simulink model "vdynblksskidpad_final"  (R2026b)
settings: Solver=ode23t  StopTime=inf  RelTol=5e-3
model workspace (MAT data in the model file):
  Eng.Tbts = [18.9199441202 18.9199441202 24.2934146345 29.2101064979 38.0525747067 43.75 43.7497238015 43.7499913003 43.75 43.75 43.75 43.75 43.75 39.375 35 30.625]
  Eng.Nbts = [0 1500 2107.14285714 2714.28571429 3321.42857143 3928.57142857 4535.71428571 5142.85714286 5750 6357.14285714 6964.28571429 7571.42857143 8178.57142857 8785.71428571 9392.85714286 10000]
  Nmtr = 11.5
  StartupTrim.BodyZ = -0.297506277079
  StartupTrim.Pitch = 0.00303068622905
  StartupTrim.TireCompression = 0.010016854716
  StartupTrim.WheelRadius = [0.290736809479 0.290736800352 0.290650131428 0.290650124633]
  SteerLim = 60
  TrackPoints = [-15 -12 -9 -6 -3 5.58745102111e-16 2.81978007367 5.36354042717 7.38228007367 8.67839071119 9.125 8.67839071119 ... (270 elements, 90x3)]
  Trans.InputShaftInertia = 0.01
  Trans.InputShaftDamping = 0.001
  Trans.FinalDrive = 3.25
  Trans.GearRatios = [-3.82 4.56 4.56 3.385 2.857 2.444 2 1]
  Trans.GearNums = [-1 0 1 2 3 4 5 6]
  Trans.Inertias = [0.032 0.007 0.032 0.025 0.0155 0.007 0.0025 0.0025]
  Trans.DampingCoeffs = [0.003 0.001 0.003 0.0025 0.002 0.001 0.001 0.001]
  Trans.Efficiencies = [0.9 0.9 0.9 0.9 0.9 0.95 0.95 0.95]
  Trans.ShiftTau = 0.02
  Ts = 0.02
  VEH.Mass = 230
  VEH.StaticNormalFrontLoad.FR = 575
  VEH.StaticNormalFrontLoad.FL = 575
  VEH.StaticNormalRearLoad.RR = 575
  VEH.StaticNormalRearLoad.RL = 322
  VEH.WheelBase = 1.7
  VEH.FrontAxlePositionfromCG = 0.75
  VEH.RearAxlePositionfromCG = 0.75
  VEH.HeightCG = 0.25
  VEH.FrontalArea = 2.11
  VEH.DragCoefficient = 0.33
  VEH.NumberOfWheelsPerAxle = 2
  VEH.PitchMomentInertia = 384.533333333
  VEH.RollMomentInertia = 86.4666666667
  VEH.YawMomentInertia = 413.2
  VEH.SteeringRatio = 18
  VEH.TrackWidth = 1.2
  VEH.SprungMass = 210
  VEH.InitialLongPosition = -15
  VEH.InitialLatPosition = 0
  VEH.InitialVertPosition = -0.2
  VEH.InitialRollAngle = 0
  VEH.InitialPitchAngle = 0
  VEH.InitialYawAngle = 0
  VEH.InitialLongVel = 0
  VEH.InitialLatVel = 0
  VEH.InitialVertVel = 0
  VEH.InitialRollRate = 0
  VEH.InitialPitchRate = 0
  VEH.InitialYawRate = 0
values from neighbouring files (symbols this model uses):
  n = size(e.Data,2)    [plot_skidpad_signals.m]
  z = tsMatrix(out.diagWheel.z)    [skidpad_settle_start.m]
undefined symbols (not defined in the file or in its folder): BdyFrm, InertFrm, magnitude
libraries: autolibsharedcoupling x11, simulink x8, sim3dlib x7, autolibshareddiff x5, autolibutils x4, sim3dautolib x3, vehdynlibtirecommon x3, sharedtransform x3, vehdynlibdriver x2, vehdynlibsteering x2, vehdynlibeom x2, vehdynlibviscommon x2
(part 1 of 5)
settings Model: Creator=The MathWorks, Inc.  LastModifiedBy=aaditya
settings SolverCC: ZeroCrossAlgorithm=Adaptive
settings OptimizationCC: ReuseModelBlockBuffer=off
settings DebuggingCC: IgnoredZcDiagnostic=none  SubsystemReferenceDiagnosticForUnitTest=warning

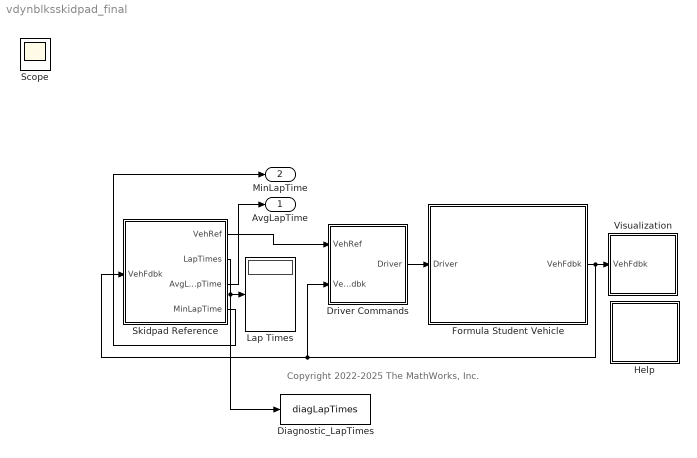
== system vdynblksskidpad_final ==
  note: Copyright 2022-2025 The MathWorks, Inc.
  Diagnostic_LapTimes : ToWorkspace  VariableName=diagLapTimes  SaveFormat=Timeseries  SampleTime=0.01
  Driver Commands : Subsystem  VariantControl=0
      mask Display: image('driverlatlongshift.png');
  Formula Student Vehicle : Subsystem  Variant=on  VariantControl=Choice  mask(Vehicle Setup){vehType=Simulink Physics}
      mask prompts: vehType "Vehicle Type:"
      mask help:
      | Choose a vehicle with powertrain and vehicle physics from Simulink blocks or one that uses a game engine physics.
      | The model will automatically configure the subsystems and settings to accomodate your choice.
      mask Help: eval('vdynblkshelp(''vdynblksformula'')');
      mask TypeOptions vehType: Game Engine Physics | Simulink Physics
      mask Callback vehType:
      | if strcmp(get_param(gcb,"vehType"),"Game Engine Physics")
      |     set_param([bdroot(gcs) '/Visualization/3D Visualization'],'engine3D','Enabled - Game Physics Vehicle')
      | else
      |     if strcmp(get_param([bdroot(gcs) '/Visualization/3D Visualization'],'engine3D'),'Enabled - Game Physics Vehicle')
      |         set_param([bdroot(gcs) '/Visualization/3D Visualization'],'engine3D','Enabled - Simulink 3D Vehicle')
      |     end
      | end
      mask Display: image('$imagefile'); % Use "Edit Image" on toolstrip to change.
  Help : Subsystem
      settings: OpenFcn=eval('vdynblkshelp(''vdynblksformula'')');
      mask Display: disp('Help')
  Lap Times : Display
  Skidpad Reference : Subsystem
      mask Display:
      | entryWidth = 3.453;
      | hOffset = 40;
      | vOffset = 15;
      | offset = [40,15];
      | entryConesLocR = [entryWidth/2 -12; entryWidth/2 -7.939];
      | entryConesLocL = [-entryWidth/2 -12;-entryWidth/2 -7.939];
      | plot(entryConesLocR(:,1)+hOffset,entryConesLocR(:,2)+vOffset);
      | plot(entryConesLocL(:,1)+hOffset,entryConesLocL(:,2)+vOffset);
      | 
      | rightInnerRingLoc = [entryWidth/2 0;...%1
      |                   4.58/2 -2.834;...%2
      |                   7.787/2 -5.231;...%3
      |                   12.588/2 -6.835;...%4
      |                   18.25/2 -7.398;...%5
      |                   23.912/2 -6.835;...%6
      |                   28.713/2 -5.231;...%7
      |                   31.92/2 -2.834;...%8
      |                   33.047/2 0;...%9
      |                   31.92/2 2.834;...%10
      |                   28.713/2 5.231;...%11
      |                   23.912/2 6.835;...%12
      |                   18.25/2 7.398;...%13
      |                   12.588/2 6.835;...%14
      |                   7.787/2 5.231;...%15
      |                   4.58/2 2.834;...%16
      |                   entryWidth/2 0;];
      | plot(rightInnerRingLoc(:,1)+hOffset,rightInnerRingLoc(:,2)+vOffset);
      | 
      | leftInnerRingLoc = rightInnerRingLoc.*[-1 1];
      | plot(leftInnerRingLoc(:,1)+hOffset,leftInnerRingLoc(:,2)+vOffset);
      | 
      | rightOutterRingLoc = [entryWidth/2 7.939;...
      |                       9.945/2 10.026;...
      |                       18.25/2 10.852;...
      |                       26.555/2 10.026;...
      |                       33.596/2 7.673;...
      |                       38.301/2 4.153;...
      |                       39.953/2 0;...
      |                       38.301/2 -4.153;...
      |                       33.596/2 -7.673;...
      |                       26.555/2 -10.026;...
      |                       18.25/2 -10.852;...
      |                       9.945/2 -10.026;...
      |                       entryWidth/2 -7.939];
      | plot(rightOutterRingLoc(:,1)+hOffset,rightOutterRingLoc(:,2)+vOffset);
      | leftOutterRingLoc = rightOutterRingLoc.*[-1 1];
      | plot(leftOutterRingLoc(:,1)+hOffset,leftOutterRingLoc(:,2)+vOffset);
      | exitConesLocL = entryConesLocL.*[1 -1];
      | exitConesLocR = entryConesLocR.*[1 -1];
      | plot(exitConesLocL(:,1)+hOffset,exitConesLocL(:,2)+vOffset);
      | plot(exitConesLocR(:,1)+hOffset,exitConesLocR(:,2)+vOffset);
      | plot([-1 1].*entryWidth/2+hOffset,[.1 .1]+vOffset)
      | plot([-1 1].*entryWidth/2+hOffset,[-.1 -.1]+vOffset)
  Visualization : Subsystem
      mask Display: disp('Visualization')
  AvgLapTime : Outport
  MinLapTime : Outport  Port=2
  Scope : Scope
      settings: ActiveDisplayYMinimum=2.1604528953399402  ActiveDisplayYMaximum=8.4344212178172668  DataLoggingVariableName=ScopeData3
  wires:
  Driver Commands/1(Driver) -> Formula Student Vehicle/1(Driver)
  Skidpad Reference/1(VehRef) -> Driver Commands/1(VehRef)
  Formula Student Vehicle/1(VehFdbk) -> Driver Commands/2(VehFdbk), Skidpad Reference/1(VehFdbk), Visualization/1(VehFdbk)
  Skidpad Reference/3(AvgLapTime) -> AvgLapTime/1
  Skidpad Reference/4(MinLapTime) -> MinLapTime/1
  Skidpad Reference/2(LapTimes) -> Lap Times/1, Diagnostic_LapTimes/1

== system vdynblksskidpad_final/Driver Commands ==
  VehRef : Inport
  VehFdbk : Inport  Port=2
  Bus Creator2 : BusCreator  Inputs=6
  Bus Selector3 : BusSelector  OutputSignals=VehFdbk.BdyFrm.Cg.Vel.xdot,VehFdbk.InertFrm.Cg.Disp.X,VehFdbk.InertFrm.Cg.Disp.Y,VehFdbk.InertFrm.Cg.Ang.psi,VehFdbk.BdyFrm.Cg.AngVel.r
  Bus Selector4 : BusSelector  OutputSignals=LngRef,PoseRef,EnblSteerCmd,SteerOvrCmd,SteerHld,SteerZero,EnblAccelOvr,AccelOvrCmd,AccelHld,AccelZero,EnblDecelCmd,DecelOvrCmd,DecelHld,DecelZero,CurvRef
  Constant1 : Constant  Value=0
  FixedDriveGear : Constant
  Ground1 : Ground
  Linear Predictive Driver : vehdynlibdriver/Predictive Driver  extAccelOvr=on  extDecelOvr=on  extAccelHld=on  extDecelHld=on  extAccelZero=on  extDecelZero=on  extSteerOvr=on  extSteerHld=on  extSteerZero=on  cntrlType=Predictive  cntrlTypeLat=Stanley  shftType=External  coordMode=SAE J670 (Z-down)  refType=Reference pose  velUnits=km/h  angUnits=rad  gearOut=on  steerOut=off  Kp=3  Ki=1  Kff=1  Kg=0  VehVelVec=[0 100]  KffVec=[.1 .1]  KpVec=[10 10]  KiVec=[5 5]  KgVec=[0 0]  vnom=5  Kaw=1  tauerr=.075  tau=.1  L=6  Kpt=8000  aR=200  bR=2.5  cR=.5  g=9.81  vecPose=on  dynamMode=on  PositionGainF=2.5  PositionGainR=.5  YawRateGain=.1  DelayGain=.01  enableDrift=off  BetaRef=10  KpBeta=1  KpDrift=1  KdDrift=1  KpPsi=1  KOmega=.1  tOmega=.1  a=VEH.FrontAxlePositionfromCG  b=VEH.RearAxlePositionfromCG  m=VEH.Mass  Cy_f=75000  Cy_r=70000  I=VEH.YawMomentInertia  Ksteer=1  theta=SteerLim*pi/180  Idl=1  Re=.3  lambda_mu=1  GearInit=1  tShift=.1  pdlVec=[0.1 0.4 0.5 0.9]  upShftTbl=[-1 12.9375 26.4375 39.9375 51.18749999999999 62.4375 72.84375 83.25;-1 16.3125 29.8125 43.3125 54.5624 65.8125 76.78125 87.75;-1 19.6875 33.1875 46.68749999999999 57.9375 69.1875 80.71875 92.25;-1 33 52.5 77.25 100.5 138.75 161.875 185]./2  dwnShftTbl=[-1 12.9375 26.4375 39.9375 51.18749999999999 62.4375 72.84375 83.25;-1 16.3125 29.8125 43.3125 54.5624 65.8125 76.78125 87.75;-1 19.6875 33.1875 46.68749999999999 57.9375 69.1875 80.71875 92.25;-1 33 52.5 77.25 100.5 138.75 161.875 185]./4  tClutch=.1  tRev=.5  tPark=120  UpGearVec="[0  1  2  3  4  5  6  7]"  DownGearVec="[1  2  3  4  5  6  7  8]"  aMode=2
  Mux1 : Mux  Inputs=3
  Mux2 : Mux  Inputs=2
  Selector1 : Selector  InputPortWidth=3  IndexOptions=Index vector (dialog)  Indices=[1 2]  OutputSizes=1  RuntimeRangeChecks=off
  Subsystem : Subsystem
  Terminator1 : Terminator
  Unit Conversion : UnitConversion
  Driver : Outport  VectorParamsAs1DForOutWhenUnconnected=off
  wires:
  Linear Predictive Driver/4 -> Bus Creator2/3, Subsystem/1(DecelCmd)  "DecelCmd"
  Linear Predictive Driver/2 -> Bus Creator2/1  "SteerCmd"
  Bus Creator2/1 -> Driver/1
  Linear Predictive Driver/3 -> Bus Creator2/2  "AccelCmd"
  Linear Predictive Driver/5 -> Bus Creator2/4, Subsystem/2(GearCmd)  "GearCmd"
  Bus Selector4/9 -> Linear Predictive Driver/9  "<AccelHld>"
  Bus Selector3/1 -> Unit Conversion/1  "<xdot>"
  Bus Selector4/13 -> Linear Predictive Driver/13  "<DecelHld>"
  Bus Selector4/14 -> Linear Predictive Driver/14  "<DecelZero>"
  Bus Selector4/7 -> Linear Predictive Driver/7  "<EnblAccelOvr>"
  Bus Selector4/11 -> Linear Predictive Driver/11  "<EnblDecelCmd>"
  Bus Selector4/1 -> Linear Predictive Driver/1  "<LngRef>"
  Bus Selector4/12 -> Linear Predictive Driver/12  "<DecelOvrCmd>"
  Bus Selector4/8 -> Linear Predictive Driver/8  "<AccelOvrCmd>"
  Bus Selector4/4 -> Linear Predictive Driver/4  "<SteerOvrCmd>"
  Bus Selector4/10 -> Linear Predictive Driver/10  "<AccelZero>"
  Bus Selector4/5 -> Linear Predictive Driver/5  "<SteerHld>"
  Bus Selector4/6 -> Linear Predictive Driver/6  "<SteerZero>"
  Bus Selector4/3 -> Linear Predictive Driver/3  "<EnblSteerCmd>"
  Linear Predictive Driver/1 -> Terminator1/1
  VehFdbk/1 -> Bus Selector3/1
  VehRef/1 -> Bus Selector4/1
  Bus Selector3/4 -> Mux1/3  "<psi>"
  Bus Selector3/2 -> Mux1/1  "<X>"
  Bus Selector3/3 -> Mux1/2  "<Y>"
  Subsystem/1(Light controls) -> Bus Creator2/5  "Light controls"
  Bus Selector4/2 -> Linear Predictive Driver/2, [PoseRef]  "<PoseRef>"
  Mux1/1 -> Linear Predictive Driver/19  "Ref"
  Selector1/1 -> Mux2/1
  [PoseRef] -> Selector1/1
  Constant1/1 -> Mux2/2
  Mux2/1 -> Bus Creator2/6  "Ref"
  Unit Conversion/1 -> Linear Predictive Driver/18
  Bus Selector4/15 -> Linear Predictive Driver/17  "<CurvRef>"
  Bus Selector3/5 -> Linear Predictive Driver/20  "<r>"
  Ground1/1 -> Linear Predictive Driver/16
  FixedDriveGear/1 -> Linear Predictive Driver/15

== system vdynblksskidpad_final/Formula Student Vehicle ==
  Driver : Inport
  Game Engine Physics : Subsystem  VariantControl=vehType==1
  Simulink Physics - 7DOF : Subsystem  VariantControl=vehType==2
  VehFdbk : Outport

== system vdynblksskidpad_final/Help ==

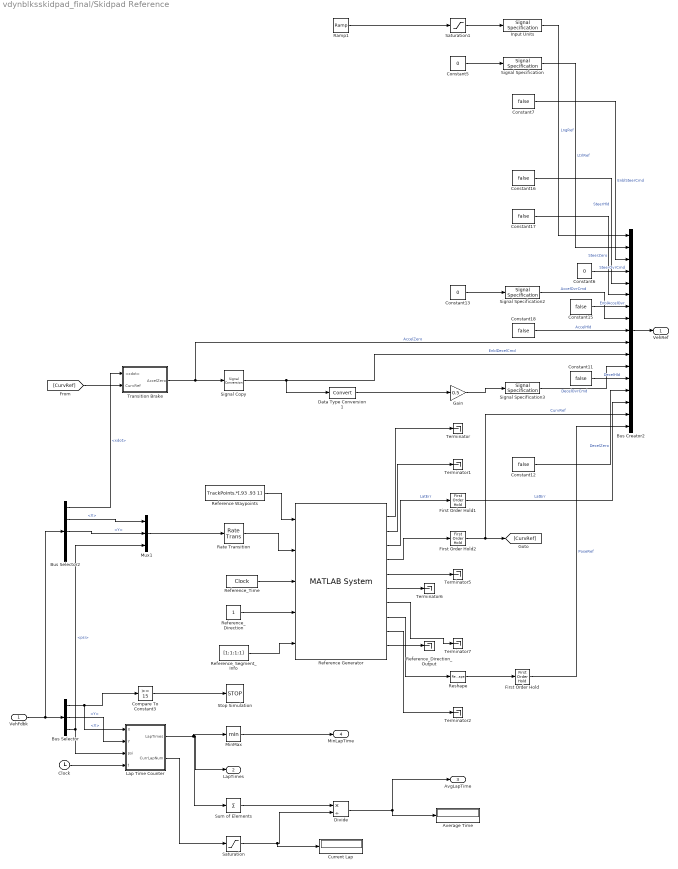
== system vdynblksskidpad_final/Skidpad Reference ==
  VehFdbk : Inport
  Average Time : Display
  Bus Creator2 : BusCreator  Inputs=17
  Bus Selector : BusSelector  OutputSignals=VehFdbk.InertFrm.Cg.Disp.X,VehFdbk.InertFrm.Cg.Disp.Y,VehFdbk.InertFrm.Cg.Ang.psi
  Bus Selector2 : BusSelector  OutputSignals=VehFdbk.BdyFrm.Cg.Vel.xdot,VehFdbk.InertFrm.Cg.Disp.X,VehFdbk.InertFrm.Cg.Disp.Y,VehFdbk.InertFrm.Cg.Vel.Xdot,VehFdbk.InertFrm.Cg.Vel.Ydot
  Clock : Clock
  Compare To Constant3 : simulink/Logic and Bit Operations/Compare To Constant  relop=>=  const=15  OutDataTypeStr=boolean  ZeroCross=off
  Constant{11..12,15..18} (6 alike) : Constant  Value=false
  Constant13 : Constant  Value=0
  Constant5 : Constant  Value=0
  Constant6 : Constant  Value=0
  Constant7 : Constant  Value=false  OutDataTypeStr=boolean
  Current Lap : Display
  Data Type Conversion1 : DataTypeConversion  SaturateOnIntegerOverflow=off  RndMeth=Floor
  Divide : Product  Inputs=*/
  First Order Hold : FirstOrderHold  InitialOutput=[VEH.InitialLongPosition VEH.InitialLatPosition VEH.InitialYawAngle]  ErrorTolerance=.1
  First Order Hold1 : FirstOrderHold  ErrorTolerance=.1
  First Order Hold2 : FirstOrderHold  ErrorTolerance=.1
  Gain : Gain  Gain=0.5
  Input Units : SignalSpecification  Unit=km/h
  Lap Time Counter : MATLAB Function  TreatAsAtomicUnit=on
  MinMax : MinMax
  Mux1 : Mux  Inputs=3
  Ramp1 : simulink/Sources/Ramp  slope=5  start=2  InitialOutput=0
  Rate Transition : RateTransition  InitialCondition=[VEH.InitialLongPosition; VEH.InitialLatPosition; VEH.InitialYawAngle]  OutPortSampleTime=Ts
  Reference Generator : vehdynlibdriver/Predictive Driver/Pose Routing/XY Waypoints Vector/MATLAB System  ShowRefPath=off  numOfHrzPoints=20  RollingSegment=off  SegLen=1000  arcLengthHorizon=10  LoopTrajectory=off  SimulateUsing=Interpreted execution
  Reference Waypoints : Constant  Value=TrackPoints.*[.93 .93 1]
  Reference_Direction : Constant
  Reference_Direction_Output : Terminator
  Reference_Segment_Info : Constant  Value=[1;1;1;1]
  Reference_Time : DigitalClock  SampleTime=Ts
  Reshape : Reshape
  Saturation : Saturate  UpperLimit=6  LowerLimit=1  ZeroCross=off
  Saturation1 : Saturate  UpperLimit=39.0  LowerLimit=0  ZeroCross=off
  Signal Copy : SignalConversion  OverrideOpt=off
  Signal Specification : SignalSpecification  Unit=m
  Signal Specification2 : SignalSpecification  Unit=one
  Signal Specification3 : SignalSpecification  Unit=one
  Stop Simulation : Stop
  Sum of Elements : Sum  Inputs=+
  Terminator{,1..2,5..7} (6 alike) : Terminator
  Transition Brake : Subsystem
  VehRef : Outport
  LapTimes : Outport  Port=2
  AvgLapTime : Outport  Port=3
  MinLapTime : Outport  Port=4
  wires:
  Reference Generator/10 -> Reference_Direction_Output/1
  Reference_Segment_Info/1 -> Reference Generator/5
  Reference_Direction/1 -> Reference Generator/4
  Reference_Time/1 -> Reference Generator/3
  MinMax/1 -> MinLapTime/1
  [CurvRef] -> Transition Brake/2(CurvRef)
  Saturation/1 -> Divide/2, Current Lap/1
  Divide/1 -> Average Time/1, AvgLapTime/1
  Sum of Elements/1 -> Divide/1
  Lap Time Counter/2(CurrLapNum) -> Saturation/1
  Compare To Constant3/1 -> Stop Simulation/1
  Bus Selector2/1 -> Transition Brake/1(<xdot>)  "<xdot>"
  Transition Brake/1(AccelZero) -> Bus Creator2/10, Signal Copy/1  "AccelZero"
  First Order Hold2/1 -> Bus Creator2/16, [CurvRef]  "CurvRef"
  Reference Generator/3 -> First Order Hold1/1  "LatErr"
  First Order Hold/1 -> Bus Creator2/17  "PoseRef"
  Rate Transition/1 -> Reference Generator/2
  Gain/1 -> Signal Specification3/1
  Data Type Conversion1/1 -> Gain/1
  Reference Waypoints/1 -> Reference Generator/1
  Lap Time Counter/1(LapTimes) -> Sum of Elements/1, LapTimes/1, MinMax/1
  Clock/1 -> Lap Time Counter/4(t)
  Bus Selector/3 -> Mux1/3, Lap Time Counter/3(psi)  "<psi>"
  Bus Selector/2 -> Lap Time Counter/2(Y)  "<Y>"
  Bus Selector/1 -> Lap Time Counter/1(X), Compare To Constant3/1  "<X>"
  Reshape/1 -> First Order Hold/1
  Bus Selector2/3 -> Mux1/2  "<Y>"
  Mux1/1 -> Rate Transition/1
  Bus Selector2/2 -> Mux1/1  "<X>"
  Constant6/1 -> Bus Creator2/4  "SteerOvrCmd"
  Constant15/1 -> Bus Creator2/7  "EnblAccelOvr"
  Constant12/1 -> Bus Creator2/14  "DecelZero"
  Reference Generator/1 -> Terminator/1
  Signal Specification3/1 -> Bus Creator2/12  "DecelOvrCmd"
  Signal Specification2/1 -> Bus Creator2/8  "AccelOvrCmd"
  Constant18/1 -> Bus Creator2/9  "AccelHld"
  Ramp1/1 -> Saturation1/1
  Bus Creator2/1 -> VehRef/1
  Input Units/1 -> Bus Creator2/1  "LngRef"
  First Order Hold1/1 -> Bus Creator2/15  "LatErr"
  Reference Generator/9 -> Terminator2/1
  Constant17/1 -> Bus Creator2/6  "SteerZero"
  Constant5/1 -> Signal Specification/1
  Signal Copy/1 -> Bus Creator2/11, Data Type Conversion1/1  "EnblDecelCmd"
  VehFdbk/1 -> Bus Selector2/1, Bus Selector/1
  Constant16/1 -> Bus Creator2/5  "SteerHld"
  Reference Generator/6 -> Terminator6/1
  Reference Generator/4 -> First Order Hold2/1
  Reference Generator/2 -> Terminator1/1
  Reference Generator/5 -> Terminator5/1
  Reference Generator/8 -> Reshape/1
  Reference Generator/7 -> Terminator7/1
  Constant11/1 -> Bus Creator2/13  "DecelHld"
  Constant7/1 -> Bus Creator2/3  "EnblSteerCmd"
  Signal Specification/1 -> Bus Creator2/2  "LtrlRef"
  Constant13/1 -> Signal Specification2/1
  Saturation1/1 -> Input Units/1

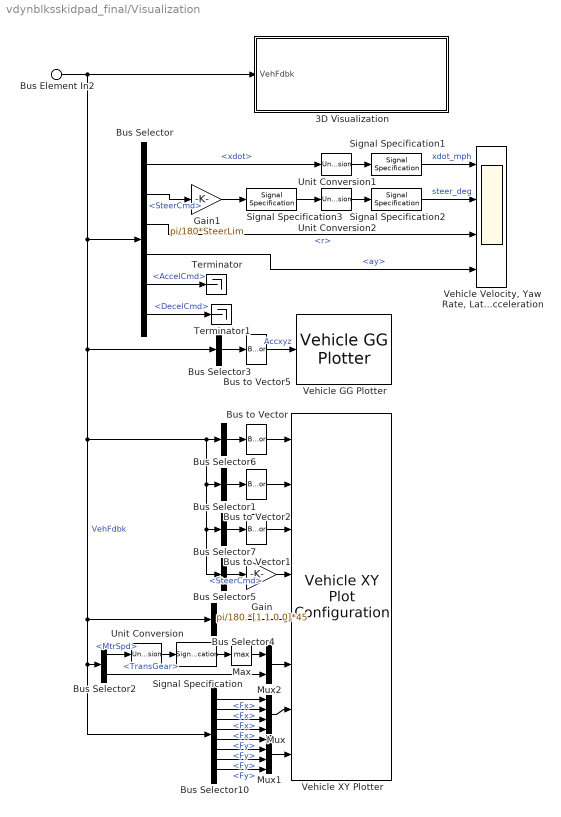
== system vdynblksskidpad_final/Visualization ==
  Bus Element In2 : Inport  PortName=VehFdbk
  3D Visualization : Subsystem  Variant=on  VariantControl=Choice  mask(3D Visualization Setup){engine3D=Disabled, conesOn=off, annotOn=off, pathOn=off, InitialPos=[ VEH.InitialLongPosition, VEH.InitialLatPosition, VEH.InitialVertPosition ], InitialRot=[VEH.InitialRollAngle VEH.InitialPitchAngle VEH.InitialYawAngle], Ts=Ts}
      mask prompts: engine3D "Visualization Mode:"; conesOn "Include cones"; annotOn "Include annotations"; pathOn "Include path markers"; InitialPos "shared_sim3dblks:sim3dblkVehicleWithGroundFollowingVDBS:blkPrm_InitialPos"; InitialRot "shared_sim3dblks:sim3dblkVehicleWithGroundFollowingVDBS:blkPrm_InitialRotSAE"; Ts "shared_sim3dblks:sim3dblkConfig:Ts"
      mask help: This is an example specific block designed to only work with vydnblksskidpad.slx. It is used in conjuction with the vehicle subystem to provide options for the 3D game engine visualization (requires Simulink 3D Animation).
      mask init:
      | visType = get_param(gcb,"engine3D");
      | switch visType
      |     case "Disabled"
      |         autoblksenableparameters(gcb, [],{'conesOn';'annotOn';'pathOn'},[],[],true);
      |         set_param([bdroot '/Formula Student Vehicle'],'vehType','Simulink Physics')
      |     case "Enabled - Ground Following Vehicle"
      |         set_param([bdroot '/Formula Student Vehicle'],'vehType','Simulink Physics')
      |         autoblksenableparameters(gcb, {'conesOn';'annotOn';'pathOn'},[],[],[],true);
      |     case "Enabled - Game Physics Vehicle"
      |         set_param([bdroot '/Formula Student Vehicle'],'vehType','Game Engine Physics')
      |         autoblksenableparameters(gcb, {'conesOn';'annotOn';'pathOn'},[],[],[],true);
      | end
      settings: AttributesFormatString=%<engine3D>
      mask TypeOptions engine3D: Disabled | Enabled - Simulink 3D Vehicle | Enabled - Game Physics Vehicle
      mask Callback engine3D:
      | if strcmp(get_param(gcb,"engine3D"),"Disabled")
      |     autoblksenableparameters(gcb, [],{'conesOn';'annotOn';'pathOn'},[],[],true);
      | else
      |     autoblksenableparameters(gcb, {'conesOn';'annotOn';'pathOn'},[],[],[],true);
      | end
      mask DialogControl InitialPos Prompt: Initial position [X, Y, Z], InitialPos:
      mask DialogControl InitialRot Prompt: Initial rotation [Roll, Pitch, Yaw], InitialRot:
      mask DialogControl Ts Prompt: Sample time:
  Bus Selector : BusSelector  OutputSignals=VehFdbk.BdyFrm.Cg.Vel.xdot,Driver.SteerCmd,VehFdbk.BdyFrm.Cg.AngVel.r,VehFdbk.BdyFrm.Cg.Acc.ay,Driver.AccelCmd,Driver.DecelCmd
  Bus Selector1 : BusSelector  OutputSignals=VehFdbk.InertFrm.Cg.Ang.phi,VehFdbk.InertFrm.Cg.Ang.theta,VehFdbk.InertFrm.Cg.Ang.psi  OutputAsBus=on
  Bus Selector10 : BusSelector  OutputSignals=VehFdbk.BdyFrm.Forces.Tires.FrntTires.Lft.Fx,VehFdbk.BdyFrm.Forces.Tires.FrntTires.Rght.Fx,VehFdbk.BdyFrm.Forces.Tires.RearTires.Lft.Fx,VehFdbk.BdyFrm.Forces.Tires.RearTires.Rght.Fx,VehFdbk.BdyFrm.Forces.Tires.FrntTires.Lft.Fy,VehFdbk.BdyFrm.Forces.Tires.FrntTires.Rght.Fy,VehFdbk.BdyFrm.Forces.Tires.RearTires.Lft.Fy,VehFdbk.BdyFrm.Forces.Tires.RearTires.Rght.Fy
  Bus Selector2 : BusSelector  OutputSignals=VehFdbk.Mtr.MtrSpd,VehFdbk.Trans.TransGear
  Bus Selector3 : BusSelector  OutputSignals=VehFdbk.BdyFrm.Cg.Acc.ax,VehFdbk.BdyFrm.Cg.Acc.ay,VehFdbk.BdyFrm.Cg.Acc.az  OutputAsBus=on
  Bus Selector4 : BusSelector  OutputSignals=Driver.Ref  OutputAsBus=on
  Bus Selector5 : BusSelector  OutputSignals=Driver.SteerCmd
  Bus Selector6 : BusSelector  OutputSignals=VehFdbk.InertFrm.Cg.Disp.X,VehFdbk.InertFrm.Cg.Disp.Y,VehFdbk.InertFrm.Cg.Disp.Z  OutputAsBus=on
  Bus Selector7 : BusSelector  OutputSignals=VehFdbk.InertFrm.Cg.Vel.Xdot,VehFdbk.InertFrm.Cg.Vel.Ydot,VehFdbk.InertFrm.Cg.Vel.Zdot  OutputAsBus=on
  Bus to Vector{,1..2,5} (4 alike) : BusToVector
  Gain : Gain  Gain=pi/180.*[1 1 0 0]*45
  Gain1 : Gain  Gain=pi/180*SteerLim
  Max : MinMax  Function=max  ZeroCross=off
  Mux : Mux
  Mux1 : Mux
  Mux2 : Mux  Inputs=2
  Signal Specification : SignalSpecification  Unit=rad/s
  Signal Specification1 : SignalSpecification  Unit=mph
  Signal Specification2 : SignalSpecification  Unit=deg
  Signal Specification3 : SignalSpecification  Unit=rad
  Terminator : Terminator
  Terminator1 : Terminator
  Unit Conversion : UnitConversion
  Unit Conversion1 : UnitConversion
  Unit Conversion2 : UnitConversion
  Vehicle GG Plotter : vehdynlibviscommon/Vehicle GG Plotter  EnablePlotter=Plot during simulation  axesType=+z down, inertial  gScale=2  showEnvelope=off  dt=.1
  "Vehicle Velocity, Yaw Rate, Lateral Acceleration" : Scope  NumInputPorts=4
      settings: ActiveDisplayYMinimum=-3.35522  ActiveDisplayYMaximum=27.7947
  Vehicle XY Plotter : vehdynlibviscommon/Vehicle XY Plot Configuration  extRef=on  extStats=on  extTireF=on  a=VEH.FrontAxlePositionfromCG  b=VEH.RearAxlePositionfromCG  w=VEH.TrackWidth  figBorder=10  bufferSize=2048  velNorm=10  tireFNorm=1000  tireFMin=20  pltDT=.2
  wires:
  Bus Selector7/1 -> Bus to Vector1/1
  Bus to Vector/1 -> Vehicle XY Plotter/1
  Bus Selector6/1 -> Bus to Vector/1
  Bus to Vector1/1 -> Vehicle XY Plotter/3
  Bus Selector1/1 -> Bus to Vector2/1
  Bus Element In2/1 -> 3D Visualization/1(VehFdbk), Bus Selector3/1, Bus Selector10/1, Bus Selector2/1, Bus Selector4/1, Bus Selector5/1, Bus Selector7/1, Bus Selector1/1, Bus Selector6/1, Bus Selector/1  "VehFdbk"
  Bus to Vector2/1 -> Vehicle XY Plotter/2
  Bus Selector5/1 -> Gain/1  "<SteerCmd>"
  Unit Conversion1/1 -> Signal Specification1/1
  Bus Selector/4 -> "Vehicle Velocity, Yaw Rate, Lateral Acceleration"/4  "<ay>"
  Bus Selector/1 -> Unit Conversion1/1  "<xdot>"
  Signal Specification1/1 -> "Vehicle Velocity, Yaw Rate, Lateral Acceleration"/1  "xdot_mph"
  Bus Selector/3 -> "Vehicle Velocity, Yaw Rate, Lateral Acceleration"/3  "<r>"
  Bus Selector4/1 -> Vehicle XY Plotter/5
  Gain/1 -> Vehicle XY Plotter/4
  Mux2/1 -> Vehicle XY Plotter/6
  Bus Selector2/2 -> Mux2/2  "<TransGear>"
  Bus Selector/2 -> Gain1/1  "<SteerCmd>"
  Unit Conversion2/1 -> Signal Specification2/1
  Signal Specification2/1 -> "Vehicle Velocity, Yaw Rate, Lateral Acceleration"/2  "steer_deg"
  Bus to Vector5/1 -> Vehicle GG Plotter/1  "Accxyz"
  Bus Selector3/1 -> Bus to Vector5/1
  Mux/1 -> Vehicle XY Plotter/7
  Mux1/1 -> Vehicle XY Plotter/8
  Bus Selector10/1 -> Mux/1  "<Fx>"
  Bus Selector10/2 -> Mux/2  "<Fx>"
  Bus Selector10/3 -> Mux/3  "<Fx>"
  Bus Selector10/4 -> Mux/4  "<Fx>"
  Bus Selector10/5 -> Mux1/1  "<Fy>"
  Bus Selector10/6 -> Mux1/2  "<Fy>"
  Bus Selector10/7 -> Mux1/3  "<Fy>"
  Bus Selector10/8 -> Mux1/4  "<Fy>"
  Gain1/1 -> Signal Specification3/1
  Signal Specification3/1 -> Unit Conversion2/1
  Unit Conversion/1 -> Signal Specification/1
  Bus Selector2/1 -> Unit Conversion/1  "<MtrSpd>"
  Signal Specification/1 -> Max/1
  Bus Selector/5 -> Terminator/1  "<AccelCmd>"
  Bus Selector/6 -> Terminator1/1  "<DecelCmd>"
  Max/1 -> Mux2/1

== system vdynblksskidpad_final/Driver Commands/Subsystem ==
  note: Light Logic
  DecelCmd : Inport
  GearCmd : Inport  Port=2
  Brake : simulink/Logic and Bit Operations/Compare To Constant  relop=>  const=.01  OutDataTypeStr=boolean  ZeroCross=off
  Highbeam : Constant  Value=false
  Left Signal : Constant  Value=false
  Lowbeam : Constant  Value=false
  Mux1 : Mux  Inputs=6
  Reverse : simulink/Logic and Bit Operations/Compare To Constant  relop=<  const=0  OutDataTypeStr=boolean  ZeroCross=off
  Right Signal : Constant  Value=false
  Light controls : Outport
  wires:
  Brake/1 -> Mux1/3
  DecelCmd/1 -> Brake/1
  Highbeam/1 -> Mux1/1
  Right Signal/1 -> Mux1/6
  Left Signal/1 -> Mux1/5
  Lowbeam/1 -> Mux1/2
  Reverse/1 -> Mux1/4
  Mux1/1 -> Light controls/1
  GearCmd/1 -> Reverse/1

== system vdynblksskidpad_final/Formula Student Vehicle/Game Engine Physics ==
  note: Vehicle Dynamics - Game Engine Physics
      | This block provides a signal and parameter interface such that a complete vehicle can be simulated and visualized with the game engine, including rigid body collision and ground contact.
  Driver : Inport
  Bus Assignment : BusAssignment  AssignedSignals=BdyFrm.Cg.Vel.xdot,InertFrm.Cg.Disp.X,InertFrm.Cg.Disp.Y,InertFrm.Cg.Ang.psi
  Bus Creator : BusCreator  Inputs=2
  Bus Selector : BusSelector  OutputSignals=SteerCmd,AccelCmd,DecelCmd,GearCmd,Light controls
  Bus Selector1 : BusSelector  OutputSignals=BdyFrm.Cg.Vel.xdot,InertFrm.Cg.Disp.X,InertFrm.Cg.Disp.Y,InertFrm.Cg.Ang.psi
  First Order Hold : FirstOrderHold  ErrorTolerance=.1
  First Order Hold1 : FirstOrderHold  InitialOutput=VEH.InitialLongPosition  ErrorTolerance=.1
  First Order Hold2 : FirstOrderHold  InitialOutput=VEH.InitialLatPosition  ErrorTolerance=.1
  First Order Hold6 : FirstOrderHold  InitialOutput=VEH.InitialYawAngle  ErrorTolerance=.01
  Rate Transition : RateTransition
  Simulation 3D Physics Vehicle : sim3dautolib/Simulation 3D Physics Vehicle  Priority=-1  PassVehMesh=Formula student vehicle  VehColor=Red  ActorName=SimulinkVehicle2  MeshPath=/MathWorksSimulation/Vehicles/Muscle/Meshes/SK_MuscleCar.SK_Sedan  TrackWidth=2  WheelBase=3  FrntWhlRadius=0.30  RearWhlRadius=0.30  FrntWhlWidth=0.20  RearWhlWidth=0.20  InitialPos=[ VEH.InitialLongPosition, VEH.InitialLatPosition, VEH.InitialVertPosition]  InitialRot=[VEH.InitialRollAngle VEH.InitialPitchAngle VEH.InitialYawAngle]  Mass=258  CgOffset=[ -.1, -.11, 0 ]  IvehScale=[1 1 1]  ChassisHeight=0.3  Cd=1.8  Cl=0.1  TrqCrv=Eng.Tbts  SpdCrv=Eng.Nbts  MaxRPM=max(Eng.Nbts)  Jmot=.02  bEngMax=.025  bEngMin=.05  DrivetrainType=Rear Wheel Drive  FrontRearSplit=0.5  TransType=Manual  G=Trans.GearNums  N=Trans.GearRatios  UpShiftRPM=4000  DownShiftRPM=2000  MinRPM=750  tShift=.02  NDiff=Trans.FinalDrive  eta=0.94  SteerType=Ackermann  SteerAngleRatio=1.0  EnableFrontSteer=on  FrntWhlMaxSteer=6*pi/180*SteerLim  EnableRearSteer=off  RearWhlMaxSteer=0  SteerSpdFctTbl=[ 1,.9, .8]  SteerVehSpdBpts=[ 0, 60, 120 ]./3.6  FrntWhlMaxTrq=5  RearWhlMaxTrq=5  HndBrkEnable=off  FrntWhlHndBrkEnable=off  RearWhlHndBrkEnable=off  FrntWhlMaxHndBrkTrq=3000  RearWhlMaxHndBrkTrq=1500  FrntSuspFOffset=[0 0 0]  RearSuspFOffset=[0 0 0]  FrntSuspMaxComp=.1  RearSuspMaxComp=.1  FrntSpringPreload=200  RearSpringPreload=200  FrntSpringRate=7e3  RearSpringRate=7e3  FrntSuspMaxExt=.1  RearSuspMaxExt=.1  FrntSuspDamping=.25  RearSuspDamping=.25  FrntRollbarScaling=.5  RearRollbarScaling=.5  ABSEnable=off  TCSEnable=off  Cy_f=250e3  Cy_r=250e3  FrntSlipThreshold=.3  RearSlipThreshold=.3  FrntSkidThreshold=1.0  RearSkidThreshold=1.0  FrntSideSlipModifier=1  RearSideSlipModifier=1  ExtMu=off  lambda_mu=10  VehLightsControl=on  HeadlightColor=[ 1, 1, 1 ]  HighBeamIntensity=100000  LowBeamIntensity=60000  HighBeamConeAngle=1.22  LowBeamConeAngle=1.22  LeftHeadlightOrientation=[ 0, 0 ]  RightHeadlightOrientation=[ 0, 0 ]  BrakelightIntensity=500  ReverselightIntensity=500  SignallightIntensity=500  SignallightPeriod=1  SignalPulseWidth=50  StandardOutportEnabled=on  TransformOutportEnabled=off  SampleTime=Ts  ActorType=SimulinkVehicle  ID=2  aMode=2  ActorTag=SimulinkVehicle2  CoordinateScheme=SAE
      settings: LibrarySourceBlock=vdynlib/Vehicle Scenarios/Sim3D/Sim3D Vehicle/Components/Simulation 3D Physics Vehicle
  Terminator{,1..3} (4 alike) : Terminator
  VehFdbk : Outport
  wires:
  Driver/1 -> Bus Selector/1, Bus Creator/2  "Driver"
  Bus Creator/1 -> VehFdbk/1
  Bus Selector/2 -> Simulation 3D Physics Vehicle/2  "<AccelCmd>"
  Bus Selector/1 -> Simulation 3D Physics Vehicle/1  "<SteerCmd>"
  Bus Selector/4 -> Simulation 3D Physics Vehicle/4  "<GearCmd>"
  Bus Selector/3 -> Simulation 3D Physics Vehicle/3  "<DecelCmd>"
  Bus Assignment/1 -> Bus Creator/1  "VehFdbk"
  Simulation 3D Physics Vehicle/2 -> Terminator/1
  Simulation 3D Physics Vehicle/3 -> Terminator1/1
  Simulation 3D Physics Vehicle/4 -> Terminator2/1
  Simulation 3D Physics Vehicle/5 -> Terminator3/1
  Simulation 3D Physics Vehicle/1 -> Bus Selector1/1, Rate Transition/1
  Bus Selector1/1 -> First Order Hold/1  "<xdot>"
  Bus Selector1/2 -> First Order Hold1/1  "<X>"
  Bus Selector1/3 -> First Order Hold2/1  "<Y>"
  Rate Transition/1 -> Bus Assignment/1
  First Order Hold/1 -> Bus Assignment/2
  Bus Selector1/4 -> First Order Hold6/1  "<psi>"
  First Order Hold1/1 -> Bus Assignment/3
  First Order Hold2/1 -> Bus Assignment/4
  First Order Hold6/1 -> Bus Assignment/5
  Bus Selector/5 -> Simulation 3D Physics Vehicle/5  "<Light controls>"

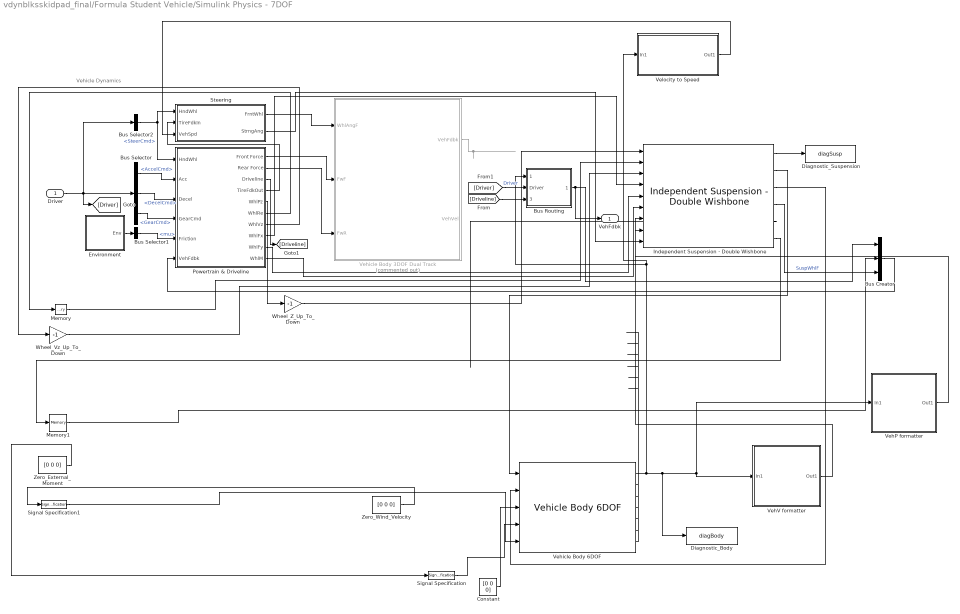
== system vdynblksskidpad_final/Formula Student Vehicle/Simulink Physics - 7DOF ==
  note: Vehicle Dynamics
  Driver : Inport
  Bus Creator : BusCreator  Inputs=3
  Bus Selector : BusSelector  OutputSignals=AccelCmd,DecelCmd,GearCmd
  Bus Selector1 : BusSelector  OutputSignals=Gnd.mu
  Bus Selector2 : BusSelector  OutputSignals=SteerCmd
  Bus Routing : Subsystem
  Constant : Constant  Value=[0 0 0]
  Diagnostic_Body : ToWorkspace  VariableName=diagBody  SaveFormat=Timeseries  SampleTime=0.01
  Diagnostic_Suspension : ToWorkspace  VariableName=diagSusp  SaveFormat=Timeseries  SampleTime=0.01
  Environment : Subsystem
      mask Display: disp('Environment')
  Independent Suspension - Double Wishbone : vehdynlibsuspension/Independent Suspension - Double Wishbone  ActiveDampEn=off  NumAxl=2  NumWhlsByAxl=[2 2]  StrgEnByAxl=[1 0]  AntiSwayEnByAxl=[0 0]  WhlNumVec="[1  2  1  2]"  AxleNumVec="[1  1  2  2]"  SuspTypesByAxle="[1  1]"  SuspImage=suspdw.png  IdealSuspEn=on  IdealSuspAxles="[1  2]"  Kz=35000  F0z=1080  Cz=2500  Hmax=0.025  f_act_susp_cz=[10000 10000;10000 10000]  f_act_susp_duty_bpt=[0 1]  f_act_susp_zdot_bpt=[-1 1]  Toe=0  RollStrgSlp=0  ToeStrgSlp=0  Caster=2.591582694*pi/180  CasterHslp=0  CasterStrgSlp=0  Camber=0  CamberHslp=0  CamberStrgSlp=0  StrgHgtSlp=0  MappedSuspEn=off  MappedSuspAxles="[1  2]"  f_susp_axl_bp=[1 2]  f_susp_dz_bp=[-0.15 -0.14 -0.13 -0.12 -0.11 -0.10 -0.09 -0.08 -0.07 -0.06 -0.05 -0.04 -0.03 -0.02 -0.01 0.00 0.01 0.02 0.03 0.04 0.05 0.06 0.07 0.08 0.09 0.10 0.11 0.12 0.13 0.14 0.15]  f_susp_dzdot_bp=[-0.15 -0.14 -0.13 -0.12 -0.11 -0.10 -0.09 -0.08 -0.07 -0.06 -0.05 -0.04 -0.03 -0.02 -0.01 0.00 0.01 0.02 0.03 0.04 0.05 0.06 0.07 0.08 0.09 0.10 0.11 0.12 0.13 0.14 0.15]  f_susp_fmz=zeros(31,31,61,2,4)  f_susp_geom=zeros(31,61,2,3)  f_susp_strgdelta_bp=[-30,-29,-28,-27,-26,-25,-24,-23,-22,-21,-20,-19,-18,-17,-16,-15,-14,-13,-12,-11,-10,-9,-8,-7,-6,-5,-4,-3,-2,-1,0,1,2,3,4,5,6,7,8,9,10,11,12,13,14,15,16,17,18,19,20,21,22,23,24,25,26,27,28,29,30]  AntiSwayR=0.2  AntiSwayNtrlAng=0.5236  AntiSwayTrsK=5.7296e+03
  Memory : Memory  InitialCondition=StartupTrim.WheelRadius
  Memory1 : Memory
  Powertrain & Driveline : Subsystem
      mask Display: image('vdbslibpt.png');
  Signal Specification : SignalSpecification  Unit=N*m
  Signal Specification1 : SignalSpecification  Unit=m/s
  Steering : Subsystem
      mask Display: image('vdbslibsteer.png');
  VehP formatter : Subsystem
  VehV formatter : Subsystem
  Vehicle Body 3DOF Dual Track : Subsystem  Commented=on
      mask Display: image('3dofdtrack.png');
  Vehicle Body 6DOF : vehdynlibeom/Vehicle Body 6DOF  extPos=on  extVel=on  extEuler=on  extRotRate=on  htchFMode=off  htchMMode=off  m=330  a=1.55*0.55  b=1.55*0.45  d=0  h=0.3  dh=1  hl=0  hh=0.1  Xe_o=[VEH.InitialLongPosition VEH.InitialLatPosition StartupTrim.BodyZ]  xbdot_o=[0,0,0]  eul_o=[0 StartupTrim.Pitch VEH.InitialYawAngle]  p_o=[0,0,0]  Iveh=[60 0 0; 0 120 0; 0 0 140]  w=[1.2,1.25]  z1m=0  z1R=[.25,.125,-0.15]  z1I=[1.4,-.2,.1;-.2,1.4,.1;.1,.1,2.25].*0  z2m=0  z2R=[-1.4,0,-0.8]  z2I=[1.4,-.2,.1;-.2,1.4,.1;.1,.1,2.25].*0  z3m=0  z3R=[-.75,-0.5,-0.4]  z3I=[5,-.1,-2;-2,9,.1;-.1,.1,6].*0  z4m=0  z4R=[-.75,.5,-0.4]  z4I=[5,-.1,-2;-2,9,.1;-.1,.1,6].*0  z5m=0  z5R=[-1.25,-.5,-0.4]  z5I=[5,-.1,-2;-2,9,.1;-.1,.1,6].*0  z6m=0  z6R=[-1.25,0.5,-0.4]  z6I=[5,-.1,-2;-2,9,.1;-.1,.1,6].*0  z7m=0  z7R=[-2,0,-0.25]  z7I=[1.4,-.2,.1;-.2,1.4,.1;.1,.1,2.25].*0  Af=1  Cd=1.8  Cl=4.8  Cpm=.1  beta_w=[0:0.001:0.01]  Cs=[0:0.01:0.1]  Cym=[0:0.001:0.01]  Pabs=101325  extTamb=off  Tair=273  g=9.81  xdot_tol=.1  longOff=0  latOff=0  vertOff=0.35  wrapAng=on  aMode=2
  Velocity to Speed : Subsystem
  Wheel_Vz_Up_To_Down : Gain  Gain=-1
  Wheel_Z_Up_To_Down : Gain  Gain=-1
  Zero_External_Moment : Constant  Value=[0 0 0]
  Zero_Wind_Velocity : Constant  Value=[0 0 0]
  VehFdbk : Outport
  wires:
  Vehicle Body 3DOF Dual Track/1(VehFdbk) -> ?
  Powertrain & Driveline/2(Rear Force) -> Vehicle Body 3DOF Dual Track/3(FwR)
  Powertrain & Driveline/1(Front Force) -> Vehicle Body 3DOF Dual Track/2(FwF)
  Bus Selector/2 -> Powertrain & Driveline/3(Decel)  "<DecelCmd>"
  Steering/1(FrntWhl) -> Vehicle Body 3DOF Dual Track/1(WhlAngF)
  Powertrain & Driveline/3(Driveline) -> [Driveline]
  Bus Selector/3 -> Powertrain & Driveline/4(GearCmd)  "<GearCmd>"
  Bus Selector2/1 -> Powertrain & Driveline/1(HndWhl), Steering/1(HndWhl)  "<SteerCmd>"
  Bus Selector/1 -> Powertrain & Driveline/2(Acc)  "<AccelCmd>"
  Driver/1 -> Bus Selector2/1, [Driver], Bus Selector/1
  Environment/1(Env) -> Bus Selector1/1
  Bus Selector1/1 -> Powertrain & Driveline/5(Friction)  "<mu>"
  [Driver] -> Bus Routing/2(Driver)  "Driver"
  [Driveline] -> Bus Routing/3(Driveline)
  Powertrain & Driveline/4(TireFdkOut) -> Steering/2(TireFdkIn)
  Independent Suspension - Double Wishbone/5 -> ?
  Vehicle Body 6DOF/2 -> ?
  Vehicle Body 6DOF/3 -> ?
  Vehicle Body 6DOF/4 -> ?
  Vehicle Body 6DOF/5 -> ?
  Vehicle Body 6DOF/6 -> ?
  Vehicle Body 6DOF/7 -> ?
  Powertrain & Driveline/5(WhlPz) -> Wheel_Z_Up_To_Down/1
  Powertrain & Driveline/7(WhlVz) -> Wheel_Vz_Up_To_Down/1
  Zero_External_Moment/1 -> Signal Specification/1
  Zero_Wind_Velocity/1 -> Signal Specification1/1
  Velocity to Speed/1(Out1) -> Steering/3(VehSpd)
  Powertrain & Driveline/6(WhlRe) -> Memory/1
  Signal Specification1/1 -> Vehicle Body 6DOF/5
  Signal Specification/1 -> Vehicle Body 6DOF/4
  Vehicle Body 6DOF/1 -> VehP formatter/1(In1), VehV formatter/1(In1), Diagnostic_Body/1, Velocity to Speed/1(In1), Bus Routing/1(VehInfo)
  Wheel_Vz_Up_To_Down/1 -> Independent Suspension - Double Wishbone/3
  Independent Suspension - Double Wishbone/2 -> Vehicle Body 6DOF/1
  Independent Suspension - Double Wishbone/3 -> Vehicle Body 6DOF/2
  Independent Suspension - Double Wishbone/6 -> Memory1/1
  Memory/1 -> Independent Suspension - Double Wishbone/2
  VehV formatter/1(Out1) -> Independent Suspension - Double Wishbone/8
  VehP formatter/1(Out1) -> Independent Suspension - Double Wishbone/7
  Independent Suspension - Double Wishbone/1 -> Diagnostic_Suspension/1
  Powertrain & Driveline/8(WhlFx) -> Independent Suspension - Double Wishbone/4
  Powertrain & Driveline/9(WhlFy) -> Independent Suspension - Double Wishbone/5
  Powertrain & Driveline/10(WhlM) -> Independent Suspension - Double Wishbone/6
  Steering/2(StrngAng) -> Independent Suspension - Double Wishbone/9
  Wheel_Z_Up_To_Down/1 -> Independent Suspension - Double Wishbone/1
  Constant/1 -> Vehicle Body 6DOF/3
  Bus Routing/1(VehFdbk) -> VehFdbk/1, Bus Creator/1
  Memory1/1 -> Bus Creator/2
  Bus Creator/1 -> Powertrain & Driveline/6(VehFdbk)
  Independent Suspension - Double Wishbone/4 -> Bus Creator/3  "SuspWhlF"

== system vdynblksskidpad_final/Skidpad Reference/Transition Brake ==
  <xdot> : Inport
  CurvRef : Inport  Port=2
  Compare To Constant : simulink/Logic and Bit Operations/Compare To Constant  relop=>=  const=120  OutDataTypeStr=boolean  ZeroCross=off
  Compare To Constant1 : simulink/Logic and Bit Operations/Compare To Constant  relop=>=  const=0  OutDataTypeStr=boolean  ZeroCross=off
  Compare To Constant2 : simulink/Logic and Bit Operations/Compare To Constant  relop=<  const=260  OutDataTypeStr=boolean  ZeroCross=off
  Compare To Constant3 : simulink/Logic and Bit Operations/Compare To Constant  relop=>  const=5  OutDataTypeStr=boolean  ZeroCross=off
  Integrator : Integrator
  Logical Operator : Logic  Inputs=4  AllPortsSameDT=off  OutDataTypeStr=boolean
  AccelZero : Outport
  wires:
  Logical Operator/1 -> AccelZero/1
  Integrator/1 -> Compare To Constant2/1, Compare To Constant/1
  Compare To Constant2/1 -> Logical Operator/2
  Compare To Constant3/1 -> Logical Operator/1
  Compare To Constant/1 -> Logical Operator/3
  Compare To Constant1/1 -> Logical Operator/4
  <xdot>/1 -> Compare To Constant3/1, Integrator/1
  CurvRef/1 -> Compare To Constant1/1

== system vdynblksskidpad_final/Visualization/3D Visualization ==
  VehFdbk : Inport
  Disabled : Subsystem  VariantControl=engine3D==1
  Enabled : Subsystem  VariantControl=engine3D~=1

== system vdynblksskidpad_final/Formula Student Vehicle/Simulink Physics - 7DOF/Bus Routing ==
  VehInfo : Inport
  Driver : Inport  Port=2
  Driveline : Inport  Port=3
  Bus Creator : BusCreator  Inputs=2
  Bus Creator17 : BusCreator  Inputs=5
  Bus Creator3 : BusCreator  Inputs=2
  Bus Creator4 : BusCreator  Inputs=2
  Bus Selector3 : BusSelector  OutputSignals=MtrTrq,MtrSpd,TransGearCmd,TransGear,Wheels
  Bus Selector4 : BusSelector  OutputSignals=InertFrm,BdyFrm
  Signal Specification : SignalSpecification  Unit=rpm
  Signal Specification1 : SignalSpecification  Unit=one
  Signal Specification3 : SignalSpecification  Unit=one
  VehFdbk : Outport
  wires:
  Bus Selector3/2 -> Signal Specification/1  "<MtrSpd>"
  Bus Creator17/1 -> Bus Creator/2  "VehFdbk"
  Bus Selector3/1 -> Bus Creator3/1  "<MtrTrq>"
  Signal Specification3/1 -> Bus Creator4/1  "TransGearCmd"
  Bus Selector4/2 -> Bus Creator17/2  "<BdyFrm>"
  Bus Selector3/3 -> Signal Specification3/1  "<TransGearCmd>"
  Bus Selector3/4 -> Signal Specification1/1  "<TransGear>"
  Bus Selector4/1 -> Bus Creator17/1  "<InertFrm>"
  Bus Creator3/1 -> Bus Creator17/3  "Mtr"
  Bus Creator4/1 -> Bus Creator17/4  "Trans"
  Signal Specification1/1 -> Bus Creator4/2  "TransGear"
  Signal Specification/1 -> Bus Creator3/2  "MtrSpd"
  VehInfo/1 -> Bus Selector4/1
  Bus Creator/1 -> VehFdbk/1
  Driver/1 -> Bus Creator/1
  Driveline/1 -> Bus Selector3/1
  Bus Selector3/5 -> Bus Creator17/5  "<Wheels>"

== system vdynblksskidpad_final/Formula Student Vehicle/Simulink Physics - 7DOF/Environment ==
  Bus Creator2 : BusCreator  Inputs=2
  Constant1 : Constant  Value=0
  Constant2 : Constant  Value=0
  Constant3 : Constant  Value=[1.3 1.3 1.3 1.3]
  Constant6 : Constant  Value=0
  Ground Feedback : Subsystem  Variant=on  VariantControlMode=label  LabelModeActiveChoice=0
  Vector Concatenate1 : Concatenate  NumInputs=3
  Env : Outport  VectorParamsAs1DForOutWhenUnconnected=off
  wires:
  Ground Feedback/1(Ground) -> Bus Creator2/2  "Gnd"
  Vector Concatenate1/1 -> Bus Creator2/1  "Wind"
  Constant2/1 -> Vector Concatenate1/2  "Y"
  Bus Creator2/1 -> Env/1
  Constant6/1 -> Vector Concatenate1/3  "Z"
  Constant1/1 -> Vector Concatenate1/1  "X"
  Constant3/1 -> Ground Feedback/1(Friction)
